simulink model "Model_pid_ff"  (R2024b)
settings: Solver=VariableStepAuto  StartTime=0.0  StopTime=25  RelTol=1e-3
PostLoadFcn:
  | addpath(fileparts(fileparts(get_param(bdroot,'FileName'))));
StartFcn:
  |    addpath(fullfile(fileparts(get_param(bdroot,'FileName')),'..','scripts'));
  |    run_and_save_deferred(bdroot, 'start');
StopFcn:
  |    addpath(fullfile(fileparts(get_param(bdroot,'FileName')),'..','scripts'));
  |    run_and_save_deferred(bdroot, 'stop');
undefined symbols (not defined in the file): k_3165_load, k_3166_load, kd_3165, kd_3166, ki_3165, ki_3166, kp_3165, kp_3166, tau_3165_load, tau_3166_load, Td_3165, Td_3166, Vc_3165, Vc_3166, w_eps, X, Y, Z
libraries: sm_lib x13, nesl_utility x5, slpidlib x2
settings Model: Creator=Student  LastModifiedBy=ricca

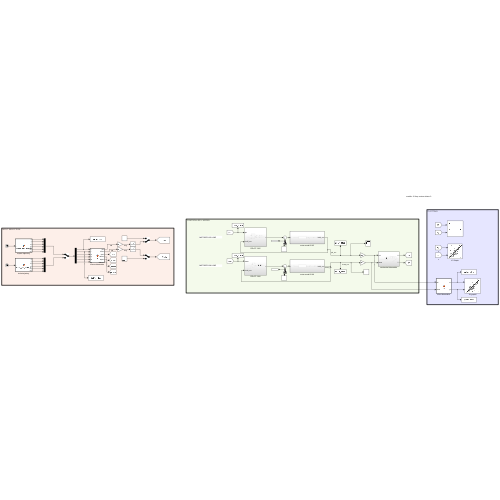
[thumbnail: Simulink's stored preview of the top-level diagram]
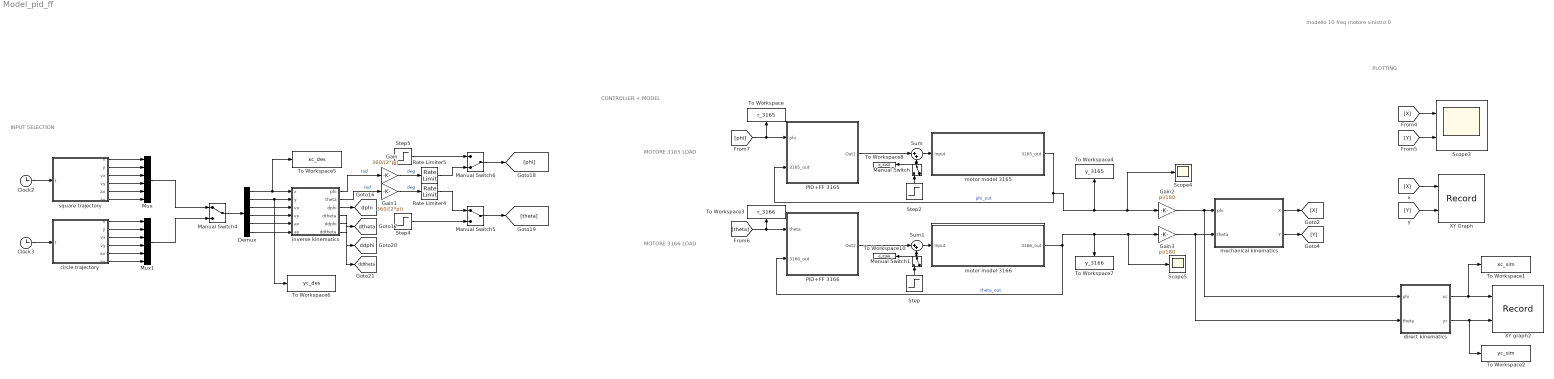
== system Model_pid_ff ==
  note: modello 10 freq motore sinistro 0
  note: PLOTTING
  note: INPUT SELECTION
  note: MOTORE 3166 LOAD
  note: CONTROLLER + MODEL
  note: MOTORE 3165 LOAD
  Clock2 : Clock
  Clock3 : Clock
  Demux : Demux  Outputs=6
  Gain : Gain  Gain=360/(2*pi)
  Gain1 : Gain  Gain=360/(2*pi)
  Gain2 : Gain  Gain=pi/180
  Gain3 : Gain  Gain=pi/180
  Manual Switch : ManualSwitch  CurrentSetting=0
  Manual Switch1 : ManualSwitch  CurrentSetting=0
  Manual Switch4 : ManualSwitch
  Manual Switch5 : ManualSwitch
  Manual Switch6 : ManualSwitch  CurrentSetting=0
  Mux : Mux  Inputs=6
  Mux1 : Mux  Inputs=6
  PID+FF 3165 : Subsystem
  PID+FF 3166 : Subsystem
  Rate Limiter4 : RateLimiter  RisingSlewLimit=100  FallingSlewLimit=-100  SampleTimeMode=inherited
  Rate Limiter5 : RateLimiter  RisingSlewLimit=100  FallingSlewLimit=-100  SampleTimeMode=inherited
  Scope3 : Scope  NumInputPorts=2
  Scope4 : Scope
  Scope5 : Scope
  Step : Step  Time=5  After=0.5  SampleTime=0
  Step2 : Step  Time=5  After=0.5  SampleTime=0
  Step4 : Step  After=10  SampleTime=0
  Step5 : Step  After=10  SampleTime=0
  Sum : Sum  Inputs=|++
  Sum1 : Sum  Inputs=|++
  To Workspace : ToWorkspace  VariableName=r_3165  SaveFormat=Timeseries  SampleTime=0.002
  To Workspace1 : ToWorkspace  VariableName=xc_sim  SaveFormat=Timeseries  SampleTime=0.002
  To Workspace10 : ToWorkspace  VariableName=d_3166  SaveFormat=Timeseries  SampleTime=-1
  To Workspace2 : ToWorkspace  VariableName=yc_sim  SaveFormat=Timeseries  SampleTime=0.002
  To Workspace3 : ToWorkspace  VariableName=r_3166  SaveFormat=Timeseries  SampleTime=0.002
  To Workspace4 : ToWorkspace  VariableName=y_3165  SaveFormat=Timeseries  SampleTime=0.002
  To Workspace5 : ToWorkspace  VariableName=xc_des  SaveFormat=Timeseries  SampleTime=0.002
  To Workspace6 : ToWorkspace  VariableName=yc_des  SaveFormat=Timeseries  SampleTime=0.002
  To Workspace7 : ToWorkspace  VariableName=y_3166  SaveFormat=Timeseries  SampleTime=0.002
  To Workspace8 : ToWorkspace  VariableName=d_3165  SaveFormat=Timeseries  SampleTime=-1
  XY Graph : Record  FileSettingsInternal="{\"entries\":[{\"content\":{\"excelSettings\":{\"content\":{},\"type\":\"Streamout.ExcelSettings\"}},\"type\":\"Streamout.FileSettingStorage\",\"uuid\":\"\"}],\"packageUris\":[\"http:\\/\\/schema.mathworks.com\\/mf0\\/streamout_blocks\\/R2020a\"],\"version\":\"1.0\"}"  Layout=[1 1]  SignalsInternal="{\"entries\":[{\"content\":{\"signals\":[{\"content\":{\"blockPath\":[],\"dimensions\":[1],\"domain\":\"\",\"lineColor\":\"#a2142f\",\"plots\":[ 1 ],\"port\":1,\"sid\":[\"\"],\"signalID\":1,\"signalName\":\"x\"},\"type\":\"RecordBlkView.Signal\",\"uuid\":\"\"},{\"content\":{\"blockPath\":[],\"dimensions\":[1],\"domain\":\"\",\"lineColor\":\"#139fff\",\"plots\":[ 1 ],\"port\":2,\"sid\":[\"\"],\"signalID\":2,\"signalName\":\"y\"},\"type\":\"RecordBlkView.Signal\",\"uuid\":\"\"}]},\"type\":\"RecordBlkView.InputSignals\",\"uuid\":\"\"}],\"packageUris\":[\"http:\\/\\/schema.mathworks.com\\/mf0\\/streamout_blocks\\/R2020a\"],\"version\":\"1.0\"}"  VisualizationBindings="{\"xyplotplugin\":{\"info\":[{\"series\":[{\"bindingParametersList\":[{\"parameter\":\"X-Axis\",\"signalID\":1,\"signalName\":\"x\"},{\"parameter\":\"Y-Axis\",\"signalID\":2,\"signalName\":\"y\"}],\"seriesID\":0}],\"subplotID\":1}]}}"  CompatibilityTag=XY
  XY graph2 : Record  FileSettingsInternal="{\"entries\":[{\"content\":{\"excelSettings\":{\"content\":{},\"type\":\"Streamout.ExcelSettings\"}},\"type\":\"Streamout.FileSettingStorage\",\"uuid\":\"\"}],\"packageUris\":[\"http:\\/\\/schema.mathworks.com\\/mf0\\/streamout_blocks\\/R2020a\"],\"version\":\"1.0\"}"  Layout=[1 1]  SignalsInternal="{\"entries\":[{\"content\":{\"signals\":[{\"content\":{\"blockPath\":[],\"dimensions\":[1],\"domain\":\"\",\"lineColor\":\"#64d413\",\"lineWidth\":2,\"port\":1,\"sid\":[\"\"],\"signalID\":1,\"signalName\":\"direct kinematics:1\"},\"type\":\"RecordBlkView.Signal\",\"uuid\":\"\"},{\"content\":{\"blockPath\":[],\"dimensions\":[1],\"domain\":\"\",\"lineColor\":\"#ff13a6\",\"lineWidth\":2,\"port\":2,\"sid\":[\"\"],\"signalID\":2,\"signalName\":\"direct kinematics:2\"},\"type\":\"RecordBlkView.Signal\",\"uuid\":\"\"}]},\"type\":\"RecordBlkView.InputSignals\",\"uuid\":\"\"}],\"packageUris\":[\"http:\\/\\/schema.mathworks.com\\/mf0\\/streamout_blocks\\/R2020a\"],\"version\":\"1.0\"}"  VisualizationBindings="{\"xyplotplugin\":{\"info\":[{\"series\":[],\"subplotID\":1}]}}"  CompatibilityTag=XY
  circle trajectory : MATLAB Function  TreatAsAtomicUnit=on
  direct kinematics : MATLAB Function  TreatAsAtomicUnit=on
  inverse kinematics : MATLAB Function  TreatAsAtomicUnit=on  SystemSampleTime=0.002
  mechanical kinematics : Subsystem
  motor model 3165 : Subsystem
  motor model 3166 : Subsystem
  square trajectory : MATLAB Function  TreatAsAtomicUnit=on
  tag scope: ddphi=global, ddtheta=global, dphi=global, dtheta=global
  wires:
  Sum/1 -> motor model 3165/1(Input)
  Sum1/1 -> motor model 3166/1(Input)
  Gain3/1 -> mechanical kinematics/2(theta), direct kinematics/2(theta)
  Rate Limiter5/1 -> Manual Switch6/2
  Demux/1 -> inverse kinematics/1(x), To Workspace5/1
  [Y] -> Scope3/2
  Manual Switch5/1 -> [theta]
  circle trajectory/6(ay) -> Mux1/6
  [Y] -> XY Graph/2
  PID+FF 3166/1(Out2) -> Sum1/1
  Clock3/1 -> circle trajectory/1(t)
  Manual Switch6/1 -> [phi]
  direct kinematics/1(xc) -> To Workspace1/1, XY graph2/1
  Mux1/1 -> Manual Switch4/2
  square trajectory/2(y) -> Mux/2
  inverse kinematics/3(dphi) -> [dphi]
  square trajectory/1(x) -> Mux/1
  Clock2/1 -> square trajectory/1(t)
  [X] -> XY Graph/1
  circle trajectory/2(y) -> Mux1/2
  inverse kinematics/4(dtheta) -> [dtheta]
  [theta] -> To Workspace3/1, PID+FF 3166/1(theta)
  square trajectory/6(ay) -> Mux/6
  Step4/1 -> Manual Switch5/2
  circle trajectory/3(vx) -> Mux1/3
  Mux/1 -> Manual Switch4/1
  inverse kinematics/1(phi) -> Gain/1  "rad"
  [phi] -> To Workspace/1, PID+FF 3165/1(phi)
  motor model 3165/1(3165_out) -> PID+FF 3165/2(3165_out), Gain2/1, Scope4/1, To Workspace4/1  "phi_out"
  circle trajectory/4(vy) -> Mux1/4
  Demux/2 -> To Workspace6/1, inverse kinematics/2(y)
  circle trajectory/5(ax) -> Mux1/5
  inverse kinematics/6(ddtheta) -> [ddtheta]
  Gain1/1 -> Rate Limiter4/1  "deg"
  motor model 3166/1(3166_out) -> PID+FF 3166/2(3166_out), To Workspace7/1, Gain3/1, Scope5/1  "theta_out"
  Gain2/1 -> direct kinematics/1(phi), mechanical kinematics/1(phi)
  inverse kinematics/2(theta) -> Gain1/1  "rad"
  inverse kinematics/5(ddphi) -> [ddphi]
  mechanical kinematics/2(Y) -> [Y]
  Step5/1 -> Manual Switch6/1
  Demux/6 -> inverse kinematics/6(ay)
  Demux/4 -> inverse kinematics/4(vy)
  Gain/1 -> Rate Limiter5/1  "deg"
  direct kinematics/2(yc) -> To Workspace2/1, XY graph2/2
  Demux/3 -> inverse kinematics/3(vx)
  square trajectory/3(vx) -> Mux/3
  circle trajectory/1(x) -> Mux1/1
  [X] -> Scope3/1
  PID+FF 3165/1(Out1) -> Sum/1
  Demux/5 -> inverse kinematics/5(ax)
  square trajectory/5(ax) -> Mux/5
  mechanical kinematics/1(X) -> [X]
  Rate Limiter4/1 -> Manual Switch5/1
  Manual Switch4/1 -> Demux/1
  square trajectory/4(vy) -> Mux/4
  Step2/1 -> Manual Switch/1
  Manual Switch/1 -> Sum/2, To Workspace8/1
  Step/1 -> Manual Switch1/1
  Manual Switch1/1 -> Sum1/2, To Workspace10/1

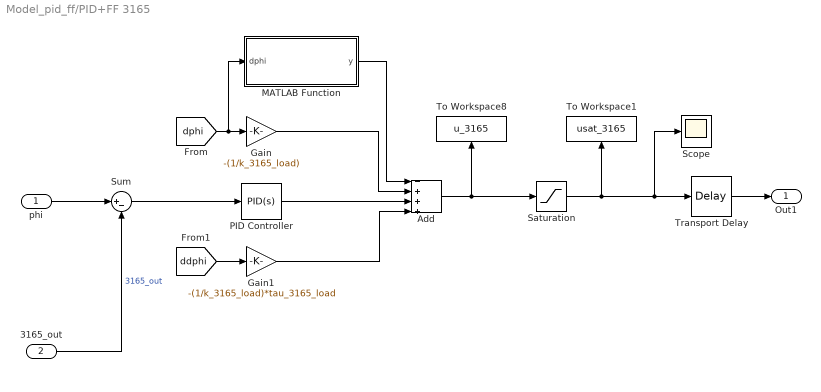
== system Model_pid_ff/PID+FF 3165 ==
  phi : Inport
  3165_out : Inport  Port=2
  Add : Sum  Inputs=-+++
  Gain : Gain  Gain=-(1/k_3165_load)
  Gain1 : Gain  Gain=-(1/k_3165_load)*tau_3165_load
  MATLAB Function : MATLAB Function  TreatAsAtomicUnit=on
  PID Controller : slpidlib/PID Controller  Controller=PID  Form=Parallel  TimeDomain=Continuous-time  UseExternalTs=off  SampleTime=-1  IntegratorMethod=Forward Euler  FilterMethod=Forward Euler  ControllerParametersSource=internal  P=kp_3165  I=ki_3165  UseKiTs=off  D=kd_3165  UseExternalDerivativeSource=off  N=100  UseFilter=on  TunerSelectOption=Transfer Function Based (PID Tuner App)  InitialConditionSource=internal  InitialConditionForIntegrator=0  InitialConditionForFilter=0  DifferentiatorICPrevScaledInput=0  ExternalReset=none  TrackingMode=off  Kt=1  LimitOutput=off  SatLimitsSource=internal  UpperSaturationLimit=inf  LowerSaturationLimit=-inf  LinearizeAsGain=on  AntiWindupMode=none  Kb=1  LimitIntegrator=off  UpperIntegratorSaturationLimit=inf  LowerIntegratorSaturationLimit=-inf  POutMin=[]  POutMax=[]  IOutMin=[]  IOutMax=[]  DOutMin=[]  DOutMax=[]  NOutMin=[]  NOutMax=[]  SumOutMin=[]  SumOutMax=[]  SaturationOutMin=[]  SaturationOutMax=[]  PParamMin=[]  PParamMax=[]  IParamMin=[]  IParamMax=[]  DParamMin=[]  DParamMax=[]  NParamMin=[]  NParamMax=[]  KbParamMin=[]  KbParamMax=[]  KtParamMin=[]  KtParamMax=[]  KbOutMin=[]  KbOutMax=[]  KtOutMin=[]  KtOutMax=[]  IntegratorOutMin=[]  IntegratorOutMax=[]  FilterOutMin=[]  FilterOutMax=[]  SumI1OutMin=[]  SumI1OutMax=[]  SumI2OutMin=[]  SumI2OutMax=[]  SumI3OutMin=[]  SumI3OutMax=[]  SumI4OutMin=[]  SumI4OutMax=[]  SumDOutMin=[]  SumDOutMax=[]  DifferentiatorOutMin=[]  DifferentiatorOutMax=[]  FilterDiffOutCoefMin=[]  FilterDiffOutCoefMax=[]  ReciprocalOutMin=[]  ReciprocalOutMax=[]  SumDenOutMin=[]  SumDenOutMax=[]  SumNumOutMin=[]  SumNumOutMax=[]  DivideOutMin=[]  DivideOutMax=[]  UdiffTsProdOutMin=[]  UdiffTsProdOutMax=[]  NTsProdOutMin=[]  NTsProdOutMax=[]  UintegralTsProdOutMin=[]  UintegralTsProdOutMax=[]  UngainTsProdOutMin=[]  UngainTsProdOutMax=[]  ClampingZeroOutDataTypeStr=Inherit: Inherit via back propagation  ClampingZeroOutMin=[]  ClampingZeroOutMax=[]  FilterDenConstantOutDataTypeStr=Inherit: Inherit via back propagation  FilterDenConstantOutMin=[]  FilterDenConstantOutMax=[]  PCopyOutDataTypeStr=Inherit: Inherit via back propagation  PCopyOutMin=[]  PCopyOutMax=[]  NCopyOutDataTypeStr=Inherit: Inherit via back propagation  NCopyOutMin=[]  NCopyOutMax=[]  IntegratorContinuousStateAttributes=''  IntegratorStateMustResolveToSignalObject=off  IntegratorRTWStateStorageClass=Auto  FilterContinuousStateAttributes=''  FilterStateMustResolveToSignalObject=off  FilterRTWStateStorageClass=Auto  ParallelPVariant=InternalParameters  IdealPVariant=Disabled  IVariant=InternalParameters  DVariant=InternalParameters  IntegratorVariant=Continuous  SatVariant=Disabled  AWVariant=Passthrough  PCopyVariant=Disabled  TRVariant=Disabled  FdbkBlocksVariant=Forward  IdealPFdbkVariant=Disabled  SatFdbkVariant=Disabled  DerivativeFilterVariant=ContFilter  NVariant=InternalParameters  NCopyVariant=Disabled  FilterICVariant=InternalICsFilter  IntegratorICVariant=InternalICs  ExternalResetVariant=Disabled  TRSumVariant=Passthrough  SumFdbkVariant=Disabled  SumVariant=Sum_PID  TsampFilterVariant=InternalTs  TsampNgainVariant=Passthrough  TsampIntegralVariant=Disabled_SignalSpec  ExternalSaturationOutDataTypeStr=Inherit: Same as second input  DerivativeSourceVariant=ErrorSignal  PreIntVariant=InternalPreInt
  Saturation : Saturate  UpperLimit=6  LowerLimit=-6
  Scope : Scope
  Sum : Sum  Inputs=|+-
  To Workspace1 : ToWorkspace  VariableName=usat_3165  SaveFormat=Timeseries  SampleTime=0.002
  To Workspace8 : ToWorkspace  VariableName=u_3165  SaveFormat=Timeseries  SampleTime=0.002
  Transport Delay : TransportDelay  DelayTime=Td_3165  PadeOrder=2
  Out1 : Outport
  wires:
  3165_out/1 -> Sum/2  "3165_out"
  [ddphi] -> Gain1/1
  phi/1 -> Sum/1
  Sum/1 -> PID Controller/1
  Add/1 -> Saturation/1, To Workspace8/1
  Saturation/1 -> Scope/1, Transport Delay/1, To Workspace1/1
  [dphi] -> MATLAB Function/1(dphi), Gain/1
  MATLAB Function/1(y) -> Add/1
  Gain/1 -> Add/2
  PID Controller/1 -> Add/3
  Gain1/1 -> Add/4
  Transport Delay/1 -> Out1/1

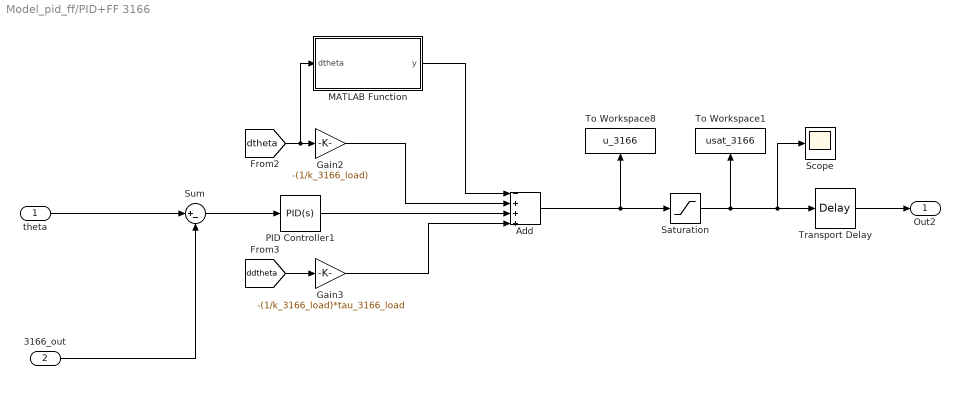
== system Model_pid_ff/PID+FF 3166 ==
  theta : Inport
  3166_out : Inport  Port=2
  Add : Sum  Inputs=-+++
  Gain2 : Gain  Gain=-(1/k_3166_load)
  Gain3 : Gain  Gain=-(1/k_3166_load)*tau_3166_load
  MATLAB Function : MATLAB Function  TreatAsAtomicUnit=on
  PID Controller1 : slpidlib/PID Controller  Controller=PID  Form=Parallel  TimeDomain=Continuous-time  UseExternalTs=off  SampleTime=-1  IntegratorMethod=Forward Euler  FilterMethod=Forward Euler  ControllerParametersSource=internal  P=kp_3166  I=ki_3166  UseKiTs=off  D=kd_3166  UseExternalDerivativeSource=off  N=100  UseFilter=on  TunerSelectOption=Transfer Function Based (PID Tuner App)  InitialConditionSource=internal  InitialConditionForIntegrator=0  InitialConditionForFilter=0  DifferentiatorICPrevScaledInput=0  ExternalReset=none  TrackingMode=off  Kt=1  LimitOutput=off  SatLimitsSource=internal  UpperSaturationLimit=inf  LowerSaturationLimit=-inf  LinearizeAsGain=on  AntiWindupMode=none  Kb=1  LimitIntegrator=off  UpperIntegratorSaturationLimit=inf  LowerIntegratorSaturationLimit=-inf  POutMin=[]  POutMax=[]  IOutMin=[]  IOutMax=[]  DOutMin=[]  DOutMax=[]  NOutMin=[]  NOutMax=[]  SumOutMin=[]  SumOutMax=[]  SaturationOutMin=[]  SaturationOutMax=[]  PParamMin=[]  PParamMax=[]  IParamMin=[]  IParamMax=[]  DParamMin=[]  DParamMax=[]  NParamMin=[]  NParamMax=[]  KbParamMin=[]  KbParamMax=[]  KtParamMin=[]  KtParamMax=[]  KbOutMin=[]  KbOutMax=[]  KtOutMin=[]  KtOutMax=[]  IntegratorOutMin=[]  IntegratorOutMax=[]  FilterOutMin=[]  FilterOutMax=[]  SumI1OutMin=[]  SumI1OutMax=[]  SumI2OutMin=[]  SumI2OutMax=[]  SumI3OutMin=[]  SumI3OutMax=[]  SumI4OutMin=[]  SumI4OutMax=[]  SumDOutMin=[]  SumDOutMax=[]  DifferentiatorOutMin=[]  DifferentiatorOutMax=[]  FilterDiffOutCoefMin=[]  FilterDiffOutCoefMax=[]  ReciprocalOutMin=[]  ReciprocalOutMax=[]  SumDenOutMin=[]  SumDenOutMax=[]  SumNumOutMin=[]  SumNumOutMax=[]  DivideOutMin=[]  DivideOutMax=[]  UdiffTsProdOutMin=[]  UdiffTsProdOutMax=[]  NTsProdOutMin=[]  NTsProdOutMax=[]  UintegralTsProdOutMin=[]  UintegralTsProdOutMax=[]  UngainTsProdOutMin=[]  UngainTsProdOutMax=[]  ClampingZeroOutDataTypeStr=Inherit: Inherit via back propagation  ClampingZeroOutMin=[]  ClampingZeroOutMax=[]  FilterDenConstantOutDataTypeStr=Inherit: Inherit via back propagation  FilterDenConstantOutMin=[]  FilterDenConstantOutMax=[]  PCopyOutDataTypeStr=Inherit: Inherit via back propagation  PCopyOutMin=[]  PCopyOutMax=[]  NCopyOutDataTypeStr=Inherit: Inherit via back propagation  NCopyOutMin=[]  NCopyOutMax=[]  IntegratorContinuousStateAttributes=''  IntegratorStateMustResolveToSignalObject=off  IntegratorRTWStateStorageClass=Auto  FilterContinuousStateAttributes=''  FilterStateMustResolveToSignalObject=off  FilterRTWStateStorageClass=Auto  ParallelPVariant=InternalParameters  IdealPVariant=Disabled  IVariant=InternalParameters  DVariant=InternalParameters  IntegratorVariant=Continuous  SatVariant=Disabled  AWVariant=Passthrough  PCopyVariant=Disabled  TRVariant=Disabled  FdbkBlocksVariant=Forward  IdealPFdbkVariant=Disabled  SatFdbkVariant=Disabled  DerivativeFilterVariant=ContFilter  NVariant=InternalParameters  NCopyVariant=Disabled  FilterICVariant=InternalICsFilter  IntegratorICVariant=InternalICs  ExternalResetVariant=Disabled  TRSumVariant=Passthrough  SumFdbkVariant=Disabled  SumVariant=Sum_PID  TsampFilterVariant=InternalTs  TsampNgainVariant=Passthrough  TsampIntegralVariant=Disabled_SignalSpec  ExternalSaturationOutDataTypeStr=Inherit: Same as second input  DerivativeSourceVariant=ErrorSignal  PreIntVariant=InternalPreInt
  Saturation : Saturate  UpperLimit=6  LowerLimit=-6
  Scope : Scope
  Sum : Sum  Inputs=|+-
  To Workspace1 : ToWorkspace  VariableName=usat_3166  SaveFormat=Timeseries  SampleTime=0.002
  To Workspace8 : ToWorkspace  VariableName=u_3166  SaveFormat=Timeseries  SampleTime=0.002
  Transport Delay : TransportDelay  DelayTime=Td_3166  PadeOrder=2
  Out2 : Outport
  wires:
  3166_out/1 -> Sum/2
  [ddtheta] -> Gain3/1
  Sum/1 -> PID Controller1/1
  [dtheta] -> MATLAB Function/1(dtheta), Gain2/1
  Add/1 -> Saturation/1, To Workspace8/1
  theta/1 -> Sum/1
  Saturation/1 -> Scope/1, Transport Delay/1, To Workspace1/1
  MATLAB Function/1(y) -> Add/1
  Gain2/1 -> Add/2
  PID Controller1/1 -> Add/3
  Gain3/1 -> Add/4
  Transport Delay/1 -> Out2/1

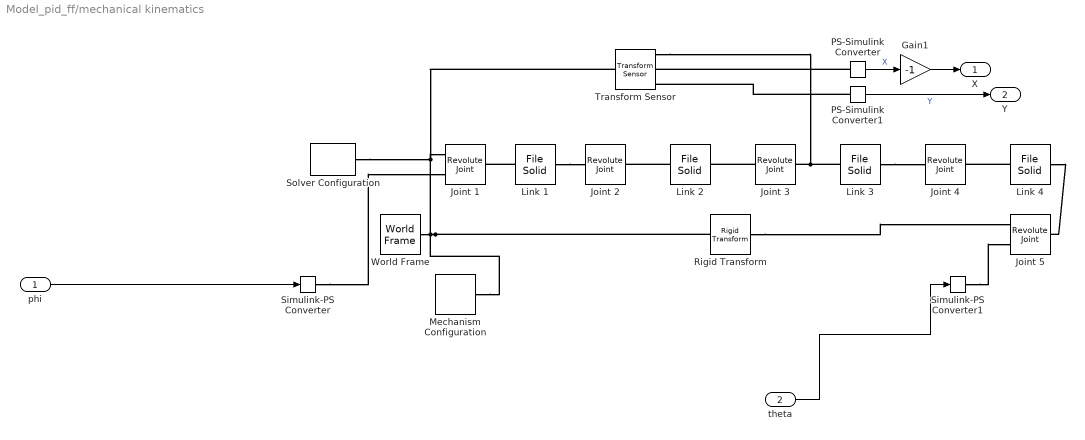
== system Model_pid_ff/mechanical kinematics ==
  phi : Inport
  theta : Inport  Port=2
  Gain1 : Gain  Gain=-1
  Joint 1 : sm_lib/Joints/Revolute Joint  JointMode=Normal  CompositeWrenchDir=FollowerOnBase  CompositeWrenchFrame=BaseFrame  SenseConstraintForce=off  SenseConstraintTorque=off  SenseTotalForce=off  SenseTotalTorque=off  PositionTargetSpecify=off  PositionTargetPriority=High  PositionTargetValue=0  PositionTargetValueUnits=deg  VelocityTargetSpecify=off  VelocityTargetPriority=High  VelocityTargetValue=0  VelocityTargetValueUnits=deg/s  EquilibriumPosition=0  EquilibriumPositionUnits=deg  SpringStiffness=0  SpringStiffnessUnits=N*m/deg  DampingCoefficient=0  DampingCoefficientUnits=N*m/(deg/s)  LowerLimitSpecify=off  LowerLimitBound=-90  LowerLimitBoundUnits=deg  LowerLimitStiffness=1e4  LowerLimitStiffnessUnits=N*m/deg  LowerLimitDamping=10  LowerLimitDampingUnits=N*m/(deg/s)  LowerLimitTransitionRegionWidth=0.1  LowerLimitTransitionRegionWidthUnits=deg  UpperLimitSpecify=off  UpperLimitBound=90  UpperLimitBoundUnits=deg  UpperLimitStiffness=1e4  UpperLimitStiffnessUnits=N*m/deg  UpperLimitDamping=10  UpperLimitDampingUnits=N*m/(deg/s)  UpperLimitTransitionRegionWidth=0.1  UpperLimitTransitionRegionWidthUnits=deg  TorqueActuationMode=ComputedTorque  MotionActuationMode=InputMotion  SensePosition=off  SenseVelocity=off  SenseAcceleration=off  SenseTorqueForce=off  SenseLowerLimitTorqueForce=off  SenseUpperLimitTorqueForce=off
  Joint 2 : sm_lib/Joints/Revolute Joint  JointMode=Normal  CompositeWrenchDir=FollowerOnBase  CompositeWrenchFrame=BaseFrame  SenseConstraintForce=off  SenseConstraintTorque=off  SenseTotalForce=off  SenseTotalTorque=off  PositionTargetSpecify=off  PositionTargetPriority=High  PositionTargetValue=90  PositionTargetValueUnits=deg  VelocityTargetSpecify=off  VelocityTargetPriority=High  VelocityTargetValue=0  VelocityTargetValueUnits=deg/s  EquilibriumPosition=0  EquilibriumPositionUnits=deg  SpringStiffness=0  SpringStiffnessUnits=N*m/deg  DampingCoefficient=0  DampingCoefficientUnits=N*m/(deg/s)  LowerLimitSpecify=off  LowerLimitBound=-90  LowerLimitBoundUnits=deg  LowerLimitStiffness=1e4  LowerLimitStiffnessUnits=N*m/deg  LowerLimitDamping=10  LowerLimitDampingUnits=N*m/(deg/s)  LowerLimitTransitionRegionWidth=0.1  LowerLimitTransitionRegionWidthUnits=deg  UpperLimitSpecify=off  UpperLimitBound=90  UpperLimitBoundUnits=deg  UpperLimitStiffness=1e4  UpperLimitStiffnessUnits=N*m/deg  UpperLimitDamping=10  UpperLimitDampingUnits=N*m/(deg/s)  UpperLimitTransitionRegionWidth=0.1  UpperLimitTransitionRegionWidthUnits=deg  TorqueActuationMode=NoTorque  MotionActuationMode=ComputedMotion  SensePosition=off  SenseVelocity=off  SenseAcceleration=off  SenseTorqueForce=off  SenseLowerLimitTorqueForce=off  SenseUpperLimitTorqueForce=off
  Joint 3 : sm_lib/Joints/Revolute Joint  JointMode=Normal  CompositeWrenchDir=FollowerOnBase  CompositeWrenchFrame=BaseFrame  SenseConstraintForce=off  SenseConstraintTorque=off  SenseTotalForce=off  SenseTotalTorque=off  PositionTargetSpecify=off  PositionTargetPriority=High  PositionTargetValue=0  PositionTargetValueUnits=deg  VelocityTargetSpecify=off  VelocityTargetPriority=High  VelocityTargetValue=0  VelocityTargetValueUnits=deg/s  EquilibriumPosition=0  EquilibriumPositionUnits=deg  SpringStiffness=0  SpringStiffnessUnits=N*m/deg  DampingCoefficient=0  DampingCoefficientUnits=N*m/(deg/s)  LowerLimitSpecify=off  LowerLimitBound=-90  LowerLimitBoundUnits=deg  LowerLimitStiffness=1e4  LowerLimitStiffnessUnits=N*m/deg  LowerLimitDamping=10  LowerLimitDampingUnits=N*m/(deg/s)  LowerLimitTransitionRegionWidth=0.1  LowerLimitTransitionRegionWidthUnits=deg  UpperLimitSpecify=off  UpperLimitBound=90  UpperLimitBoundUnits=deg  UpperLimitStiffness=1e4  UpperLimitStiffnessUnits=N*m/deg  UpperLimitDamping=10  UpperLimitDampingUnits=N*m/(deg/s)  UpperLimitTransitionRegionWidth=0.1  UpperLimitTransitionRegionWidthUnits=deg  TorqueActuationMode=NoTorque  MotionActuationMode=ComputedMotion  SensePosition=off  SenseVelocity=off  SenseAcceleration=off  SenseTorqueForce=off  SenseLowerLimitTorqueForce=off  SenseUpperLimitTorqueForce=off
  Joint 4 : sm_lib/Joints/Revolute Joint  JointMode=Normal  CompositeWrenchDir=FollowerOnBase  CompositeWrenchFrame=BaseFrame  SenseConstraintForce=off  SenseConstraintTorque=off  SenseTotalForce=off  SenseTotalTorque=off  PositionTargetSpecify=off  PositionTargetPriority=High  PositionTargetValue=0  PositionTargetValueUnits=deg  VelocityTargetSpecify=off  VelocityTargetPriority=High  VelocityTargetValue=0  VelocityTargetValueUnits=deg/s  EquilibriumPosition=0  EquilibriumPositionUnits=deg  SpringStiffness=0  SpringStiffnessUnits=N*m/deg  DampingCoefficient=0  DampingCoefficientUnits=N*m/(deg/s)  LowerLimitSpecify=off  LowerLimitBound=-90  LowerLimitBoundUnits=deg  LowerLimitStiffness=1e4  LowerLimitStiffnessUnits=N*m/deg  LowerLimitDamping=10  LowerLimitDampingUnits=N*m/(deg/s)  LowerLimitTransitionRegionWidth=0.1  LowerLimitTransitionRegionWidthUnits=deg  UpperLimitSpecify=off  UpperLimitBound=90  UpperLimitBoundUnits=deg  UpperLimitStiffness=1e4  UpperLimitStiffnessUnits=N*m/deg  UpperLimitDamping=10  UpperLimitDampingUnits=N*m/(deg/s)  UpperLimitTransitionRegionWidth=0.1  UpperLimitTransitionRegionWidthUnits=deg  TorqueActuationMode=NoTorque  MotionActuationMode=ComputedMotion  SensePosition=off  SenseVelocity=off  SenseAcceleration=off  SenseTorqueForce=off  SenseLowerLimitTorqueForce=off  SenseUpperLimitTorqueForce=off
  Joint 5 : sm_lib/Joints/Revolute Joint  JointMode=Normal  CompositeWrenchDir=FollowerOnBase  CompositeWrenchFrame=BaseFrame  SenseConstraintForce=off  SenseConstraintTorque=off  SenseTotalForce=off  SenseTotalTorque=off  PositionTargetSpecify=off  PositionTargetPriority=High  PositionTargetValue=0  PositionTargetValueUnits=deg  VelocityTargetSpecify=off  VelocityTargetPriority=High  VelocityTargetValue=0  VelocityTargetValueUnits=deg/s  EquilibriumPosition=0  EquilibriumPositionUnits=deg  SpringStiffness=0  SpringStiffnessUnits=N*m/deg  DampingCoefficient=0  DampingCoefficientUnits=N*m/(deg/s)  LowerLimitSpecify=off  LowerLimitBound=-90  LowerLimitBoundUnits=deg  LowerLimitStiffness=1e4  LowerLimitStiffnessUnits=N*m/deg  LowerLimitDamping=10  LowerLimitDampingUnits=N*m/(deg/s)  LowerLimitTransitionRegionWidth=0.1  LowerLimitTransitionRegionWidthUnits=deg  UpperLimitSpecify=off  UpperLimitBound=90  UpperLimitBoundUnits=deg  UpperLimitStiffness=1e4  UpperLimitStiffnessUnits=N*m/deg  UpperLimitDamping=10  UpperLimitDampingUnits=N*m/(deg/s)  UpperLimitTransitionRegionWidth=0.1  UpperLimitTransitionRegionWidthUnits=deg  TorqueActuationMode=ComputedTorque  MotionActuationMode=InputMotion  SensePosition=off  SenseVelocity=off  SenseAcceleration=off  SenseTorqueForce=off  SenseLowerLimitTorqueForce=off  SenseUpperLimitTorqueForce=off
  Link 1 : sm_lib/Body Elements/File Solid  ExtGeomFileName=link.step  UnitType=FromFile  ExtGeomFileUnits=m  StepReaderType=HEX  ExportConvexHullGeometry=off  InertiaType=CalculateFromGeometry  BasedOnType=Mass  Density=1000  DensityUnits=kg/m^3  Mass=0.065  MassUnits=kg  CenterOfMass=[0 0 0]  CenterOfMassUnits=m  MomentsOfInertia=[1 1 1]  MomentsOfInertiaUnits=kg*m^2  ProductsOfInertia=[0 0 0]  ProductsOfInertiaUnits=kg*m^2  GraphicType=FromGeometry  MarkerShape=Sphere  MarkerSize=10  GraphicVisPropType=SimpleVisualProperties  GraphicDiffuseColor=[0.5 0.5 0.5]  GraphicOpacity=1  GraphicSpecularColor=[0.5 0.5 0.5 1.0]  GraphicAmbientColor=[0.15 0.15 0.15 1.0]  GraphicEmissiveColor=[0.0 0.0 0.0 1.0]  GraphicShininess=75  DoExposeReferenceFrame=off  SerializedFrames=<Frames><Frame><Id>Frame1</Id><Value><Name>F1</Name><Origin><Source>GeometricFeature</Source><FeatureName>cylindrical surface 1</FeatureName></Origin><PrimaryAxis><DefinedDirection>+Z</DefinedDirection><Source>ReferenceFrame</Source><SourceDirection>+Z</SourceDirection><FeatureName></FeatureName></PrimaryAxis><SecondaryAxis><DefinedDirection>+Y</DefinedDirection><Source>ReferenceFrame</Source><SourceDirection>+X</SourceDirection><FeatureName></FeatureName></SecondaryAxis></Value></Frame><Frame><Id>Frame2</Id><Value><Name>F2</Name><Origin><Source>GeometricFeature</Source><FeatureName>cylindrical surface 2</FeatureName></Origin><PrimaryAxis><DefinedDirection>+Z</DefinedDirection><Source>ReferenceFrame</Source><SourceDirection>+Z</SourceDirection><FeatureName></FeatureName></PrimaryAxis><SecondaryAxis><DefinedDirection>+X</DefinedDirection><Source>ReferenceFrame</Source><SourceDirection>+X</SourceDirection><FeatureName></FeatureName></SecondaryAxis></Value></Frame></Frames>
  Link 2 : sm_lib/Body Elements/File Solid  ExtGeomFileName=link.step  UnitType=FromFile  ExtGeomFileUnits=m  StepReaderType=HEX  ExportConvexHullGeometry=off  InertiaType=CalculateFromGeometry  BasedOnType=Mass  Density=1000  DensityUnits=kg/m^3  Mass=0.065  MassUnits=kg  CenterOfMass=[0 0 0]  CenterOfMassUnits=m  MomentsOfInertia=[1 1 1]  MomentsOfInertiaUnits=kg*m^2  ProductsOfInertia=[0 0 0]  ProductsOfInertiaUnits=kg*m^2  GraphicType=FromGeometry  MarkerShape=Sphere  MarkerSize=10  GraphicVisPropType=SimpleVisualProperties  GraphicDiffuseColor=[0.5 0.5 0.5]  GraphicOpacity=1  GraphicSpecularColor=[0.5 0.5 0.5 1.0]  GraphicAmbientColor=[0.15 0.15 0.15 1.0]  GraphicEmissiveColor=[0.0 0.0 0.0 1.0]  GraphicShininess=75  DoExposeReferenceFrame=off  SerializedFrames=<Frames><Frame><Id>Frame1</Id><Value><Name>F1</Name><Origin><Source>GeometricFeature</Source><FeatureName>cylindrical surface 1</FeatureName></Origin><PrimaryAxis><DefinedDirection>+Z</DefinedDirection><Source>ReferenceFrame</Source><SourceDirection>+Z</SourceDirection><FeatureName></FeatureName></PrimaryAxis><SecondaryAxis><DefinedDirection>+X</DefinedDirection><Source>ReferenceFrame</Source><SourceDirection>+X</SourceDirection><FeatureName></FeatureName></SecondaryAxis></Value></Frame><Frame><Id>Frame2</Id><Value><Name>F2</Name><Origin><Source>GeometricFeature</Source><FeatureName>cylindrical surface 2</FeatureName></Origin><PrimaryAxis><DefinedDirection>+Z</DefinedDirection><Source>ReferenceFrame</Source><SourceDirection>+Z</SourceDirection><FeatureName></FeatureName></PrimaryAxis><SecondaryAxis><DefinedDirection>+X</DefinedDirection><Source>ReferenceFrame</Source><SourceDirection>+X</SourceDirection><FeatureName></FeatureName></SecondaryAxis></Value></Frame></Frames>
  Link 3 : sm_lib/Body Elements/File Solid  ExtGeomFileName=link.step  UnitType=FromFile  ExtGeomFileUnits=m  StepReaderType=HEX  ExportConvexHullGeometry=off  InertiaType=CalculateFromGeometry  BasedOnType=Mass  Density=1000  DensityUnits=kg/m^3  Mass=0.065  MassUnits=kg  CenterOfMass=[0 0 0]  CenterOfMassUnits=m  MomentsOfInertia=[1 1 1]  MomentsOfInertiaUnits=kg*m^2  ProductsOfInertia=[0 0 0]  ProductsOfInertiaUnits=kg*m^2  GraphicType=FromGeometry  MarkerShape=Sphere  MarkerSize=10  GraphicVisPropType=SimpleVisualProperties  GraphicDiffuseColor=[0.5 0.5 0.5]  GraphicOpacity=1  GraphicSpecularColor=[0.5 0.5 0.5 1.0]  GraphicAmbientColor=[0.15 0.15 0.15 1.0]  GraphicEmissiveColor=[0.0 0.0 0.0 1.0]  GraphicShininess=75  DoExposeReferenceFrame=off  SerializedFrames=<Frames><Frame><Id>Frame1</Id><Value><Name>F1</Name><Origin><Source>GeometricFeature</Source><FeatureName>cylindrical surface 1</FeatureName></Origin><PrimaryAxis><DefinedDirection>+Z</DefinedDirection><Source>ReferenceFrame</Source><SourceDirection>+Z</SourceDirection><FeatureName></FeatureName></PrimaryAxis><SecondaryAxis><DefinedDirection>+X</DefinedDirection><Source>ReferenceFrame</Source><SourceDirection>+X</SourceDirection><FeatureName></FeatureName></SecondaryAxis></Value></Frame><Frame><Id>Frame2</Id><Value><Name>F2</Name><Origin><Source>GeometricFeature</Source><FeatureName>cylindrical surface 2</FeatureName></Origin><PrimaryAxis><DefinedDirection>+Z</DefinedDirection><Source>ReferenceFrame</Source><SourceDirection>+Z</SourceDirection><FeatureName></FeatureName></PrimaryAxis><SecondaryAxis><DefinedDirection>+X</DefinedDirection><Source>ReferenceFrame</Source><SourceDirection>+X</SourceDirection><FeatureName></FeatureName></SecondaryAxis></Value></Frame></Frames>
  Link 4 : sm_lib/Body Elements/File Solid  ExtGeomFileName=link.step  UnitType=FromFile  ExtGeomFileUnits=m  StepReaderType=HEX  ExportConvexHullGeometry=off  InertiaType=CalculateFromGeometry  BasedOnType=Mass  Density=1000  DensityUnits=kg/m^3  Mass=0.065  MassUnits=kg  CenterOfMass=[0 0 0]  CenterOfMassUnits=m  MomentsOfInertia=[1 1 1]  MomentsOfInertiaUnits=kg*m^2  ProductsOfInertia=[0 0 0]  ProductsOfInertiaUnits=kg*m^2  GraphicType=FromGeometry  MarkerShape=Sphere  MarkerSize=10  GraphicVisPropType=SimpleVisualProperties  GraphicDiffuseColor=[0.5 0.5 0.5]  GraphicOpacity=1  GraphicSpecularColor=[0.5 0.5 0.5 1.0]  GraphicAmbientColor=[0.15 0.15 0.15 1.0]  GraphicEmissiveColor=[0.0 0.0 0.0 1.0]  GraphicShininess=75  DoExposeReferenceFrame=off  SerializedFrames=<Frames><Frame><Id>Frame1</Id><Value><Name>F1</Name><Origin><Source>GeometricFeature</Source><FeatureName>cylindrical surface 1</FeatureName></Origin><PrimaryAxis><DefinedDirection>+Z</DefinedDirection><Source>ReferenceFrame</Source><SourceDirection>+Z</SourceDirection><FeatureName></FeatureName></PrimaryAxis><SecondaryAxis><DefinedDirection>+X</DefinedDirection><Source>ReferenceFrame</Source><SourceDirection>+X</SourceDirection><FeatureName></FeatureName></SecondaryAxis></Value></Frame><Frame><Id>Frame2</Id><Value><Name>F2</Name><Origin><Source>GeometricFeature</Source><FeatureName>cylindrical surface 2</FeatureName></Origin><PrimaryAxis><DefinedDirection>+Z</DefinedDirection><Source>ReferenceFrame</Source><SourceDirection>+Z</SourceDirection><FeatureName></FeatureName></PrimaryAxis><SecondaryAxis><DefinedDirection>+X</DefinedDirection><Source>ReferenceFrame</Source><SourceDirection>+X</SourceDirection><FeatureName></FeatureName></SecondaryAxis></Value></Frame></Frames>
  Mechanism Configuration : sm_lib/Utilities/Mechanism Configuration  UniformGravity=Constant  GravityVector=[0 0 -9.80665]  GravityVectorUnits=m/s^2  LinearizationDelta=0.001  JointModeTransitionNonlinearIterations=2
  PS-Simulink Converter : nesl_utility/PS-Simulink Converter  PhysicalDomain=network_engine_domain  SubClassName=ps_output  LeftPortType=input  RightPortType=output  PseudoPeriodic=off  Frequencies=[]  VectorFormat=inherit  Unit=inherit  AffineConversion=off
  PS-Simulink Converter1 : nesl_utility/PS-Simulink Converter  PhysicalDomain=network_engine_domain  SubClassName=ps_output  LeftPortType=input  RightPortType=output  PseudoPeriodic=off  Frequencies=[]  VectorFormat=inherit  Unit=inherit  AffineConversion=off
  Rigid Transform : sm_lib/Frames and Transforms/Rigid Transform  RotationMethod=None  FollAlignAxisA=+X  BaseAlignAxisA=+Y  FollAlignAxisB=+Y  BaseAlignAxisB=+Z  RotationStandardAxis=+Z  RotationAngle=0  RotationAngleUnits=deg  RotationArbitraryAxis=[0 0 1]  RotationSequenceAxes=FollowerAxes  RotationSequence=XYX  RotationSequenceAngles=[0 0 0]  RotationSequenceAnglesUnits=deg  RotationMatrix=[1 0 0;0 1 0;0 0 1]  Quaternion=[1 0 0 0]  TranslationMethod=Cartesian  TranslationCartesianOffset=[0 0.254 0]  TranslationCartesianOffsetUnits=m  TranslationStandardAxis=+Z  TranslationStandardOffset=0  TranslationStandardOffsetUnits=m  TranslationROffset=0  TranslationROffsetUnits=m  TranslationThetaOffset=0  TranslationThetaOffsetUnits=deg  TranslationZOffset=0  TranslationZOffsetUnits=m
  Simulink-PS Converter : nesl_utility/Simulink-PS Converter  PhysicalDomain=network_engine_domain  SubClassName=ps_input  LeftPortType=input  RightPortType=output  PseudoPeriodic=off  Frequencies=[]  NoiseDistribution=none  NoiseParameters=[]  Unit=rad  AffineConversion=off  FilteringAndDerivatives=filter  SimscapeFilterOrder=2  InputFilterTimeConstant=0.001  UdotUserProvided=0
  Simulink-PS Converter1 : nesl_utility/Simulink-PS Converter  PhysicalDomain=network_engine_domain  SubClassName=ps_input  LeftPortType=input  RightPortType=output  PseudoPeriodic=off  Frequencies=[]  NoiseDistribution=none  NoiseParameters=[]  Unit=rad  AffineConversion=off  FilteringAndDerivatives=filter  SimscapeFilterOrder=2  InputFilterTimeConstant=0.001  UdotUserProvided=0
  Solver Configuration : nesl_utility/Solver Configuration  PhysicalDomain=network_engine_domain  SubClassName=solver  LeftPortType=input  RightPortType=generic  Tones=[]  Harmonics=[]  SimulateNoise=off  Profile=off  UseLocalSampling=off  EnableSwitchedLinearOptims=on  FrequencyDomain=off  UseCCode=off  RelTol=0.001  AbsTol=0.001  MinStep=1e-09  ToWorkspace=off  RevertToSquareIcSolve=off  NumHomotopyIterations=100  PhasorMode=off  PhasorModeNumHarmonics=1  ConsistencySolver=NEWTON_XTOL_AFTER_FTOL  IndexReductionMethod=DerivativeReplacement  DoDC=on  ResidualTolerance=1e-09  ConsistencyTolSource=GLOBAL  ConsistencyAbsTol=0.001  ConsistencyRelTol=0.001  ConsistencyTolFactor=0.001  UseLocalSolver=off  LocalSolverChoice=NE_BACKWARD_EULER_ADVANCER  ResolveIndetEquations=on  FunctionEvalNumThread=1  LocalSolverSampleTime=0.001  DoFixedCost=off  MaxNonlinIter=3  MaxModeIter=2  ComputeImpulses=off  ImpulseIterations=2  LinearAlgebra=auto  LinearAlgebraNumThread=0  EquationFormulation=NE_TIME_EF  DelaysMemoryBudget=1024  AutomaticFiltering=on  FilteringTimeConstant=0.001  PartitionStorageMethod=AS_NEEDED  PartitionMemoryBudget=1024  PartitionMethod=ROBUST  MultibodyUseLocalSolver=off  MultibodyLocalSolverChoice=ODE1  MultibodyLocalSolverSampleTime=0.001
  Transform Sensor : sm_lib/Frames and Transforms/Transform Sensor  MeasurementFrame=World  RotationSequence=XYX  SenseAngle=off  SenseAxis=off  SenseQ=off  SenseR=off  SenseRotationSequence=off  SenseOmegaX=off  SenseOmegaY=off  SenseOmegaZ=off  SenseOmega=off  SenseQDot=off  SenseRDot=off  SenseRotationSequenceDot=off  SenseAlphaX=off  SenseAlphaY=off  SenseAlphaZ=off  SenseAlpha=off  SenseQDDot=off  SenseRDDot=off  SenseX=on  SenseY=on  SenseZ=off  SenseXYZ=off  SenseRad=off  SenseAzim=off  SenseDist=off  SenseInc=off  SenseXDot=off  SenseYDot=off  SenseZDot=off  SenseXYZDot=off  SenseRadDot=off  SenseAzimDot=off  SenseDistDot=off  SenseIncDot=off  SenseXDDot=off  SenseYDDot=off  SenseZDDot=off  SenseXYZDDot=off  SenseRadDDot=off  SenseAzimDDot=off  SenseDistDDot=off  SenseIncDDot=off
  World Frame : sm_lib/Frames and Transforms/World Frame
  X : Outport
  Y : Outport  Port=2
  wires:
  theta/1 -> Simulink-PS Converter1/1
  phi/1 -> Simulink-PS Converter/1
  PS-Simulink Converter1/1 -> Y/1  "Y"
  PS-Simulink Converter/1 -> Gain1/1  "X"
  Gain1/1 -> X/1
  connections:
  World Frame/RConn1 -- Rigid Transform/LConn1 -- Transform Sensor/LConn1 -- Joint 1/LConn1 -- Solver Configuration/RConn1 -- Mechanism Configuration/RConn1
  Joint 3/LConn1 -- Link 2/RConn1
  Link 3/LConn1 -- Transform Sensor/RConn1 -- Joint 3/RConn1
  Simulink-PS Converter1/RConn1 -- Joint 5/LConn2
  Rigid Transform/RConn1 -- Joint 5/LConn1
  Link 3/RConn1 -- Joint 4/LConn1
  Link 1/RConn1 -- Joint 2/LConn1
  Link 4/LConn1 -- Joint 4/RConn1
  Link 4/RConn1 -- Joint 5/RConn1
  Link 2/LConn1 -- Joint 2/RConn1
  Link 1/LConn1 -- Joint 1/RConn1
  Simulink-PS Converter/RConn1 -- Joint 1/LConn2
  PS-Simulink Converter/LConn1 -- Transform Sensor/RConn2
  PS-Simulink Converter1/LConn1 -- Transform Sensor/RConn3

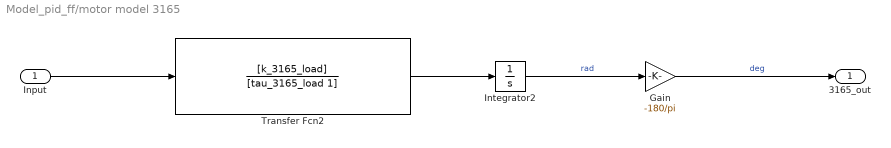
== system Model_pid_ff/motor model 3165 ==
  Input : Inport
  Gain : Gain  Gain=-180/pi
  Integrator2 : Integrator
  Transfer Fcn2 : TransferFcn  Numerator=[k_3165_load]  Denominator=[tau_3165_load 1]
  3165_out : Outport
  wires:
  Transfer Fcn2/1 -> Integrator2/1
  Input/1 -> Transfer Fcn2/1
  Integrator2/1 -> Gain/1  "rad"
  Gain/1 -> 3165_out/1  "deg"

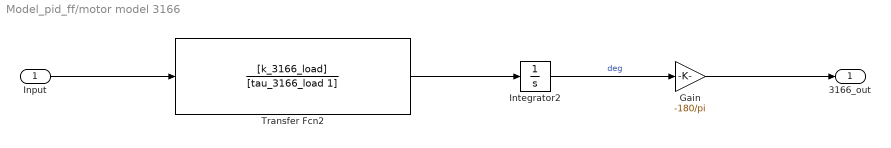
== system Model_pid_ff/motor model 3166 ==
  Input : Inport
  Gain : Gain  Gain=-180/pi
  Integrator2 : Integrator
  Transfer Fcn2 : TransferFcn  Numerator=[k_3166_load]  Denominator=[tau_3166_load 1]
  3166_out : Outport
  wires:
  Transfer Fcn2/1 -> Integrator2/1
  Input/1 -> Transfer Fcn2/1
  Integrator2/1 -> Gain/1  "deg"
  Gain/1 -> 3166_out/1

== matlab function Model_pid_ff/PID+FF 3166/MATLAB Function ==
  data: dtheta input; Vc_3166 parameter; w_eps parameter; y output
function y = friction_compensation(dtheta, Vc_3166, w_eps)
y = Vc_3166*tanh(dtheta/w_eps);

== matlab function Model_pid_ff/PID+FF 3165/MATLAB Function ==
  data: dphi input; Vc_3165 parameter; w_eps parameter; y output
function y = friction_compensation(dphi, Vc_3165, w_eps)
y = Vc_3165*tanh(dphi/w_eps);

== matlab function Model_pid_ff/direct kinematics ==
  data: phi input; xc output; theta input; yc output
function [xc, yc] = fcn(phi, theta)
l = 0.127;
a = 2 - sin(theta) - cos(phi);
b = cos(theta) - sin(phi);
s = sqrt(a^2 + b^2);
h = l*sqrt(1 - s^2/4);

% Nonlinear forward kinematics of point C
xc = l/2*(2 - sin(theta) + cos(phi)) - h*b/s;
yc = l/2*(cos(theta) + sin(phi))     + h*a/s;

== matlab function Model_pid_ff/square trajectory ==
  data: x output; t input; y output; vx output; vy output; ax output; ay output
% function [x, y, vx, vy, ax, ay] = square_gen_smooth(t)
% c  = [0.127; 0.127];
% s  = 0.09;
% T  = 4;
% Ts = T/4;
% P = [c(1)-s/2, c(1)+s/2, c(1)+s/2, c(1)-s/2, c(1)-s/2;
%      c(2)-s/2, c(2)-s/2, c(2)+s/2, c(2)+s/2, c(2)-s/2];
% 
% tau = mod(t, T) / Ts;
% k   = min(floor(tau), 3);
% f   = tau - k;
% 
% % quintic time scaling and its derivatives w.r.t. real time
% sig   = 10*f^3 - 15*f^4 + 6*f^5;
% dsig  = (30*f^2 - 60*f^3 + 30*f^4) / Ts;
% ddsig = (60*f - 180*f^2 + 120*f^3) / Ts^2;
% 
% dx = P(1,k+2) - P(1,k+1);
% dy = P(2,k+2) - P(2,k+1);
% 
% x  = P(1,k+1) + sig*dx;     y  = P(2,k+1) + sig*dy;
% vx = dsig*dx;               vy = dsig*dy;
% ax = ddsig*dx;              ay = ddsig*dy;
% end

function [x, y, vx, vy, ax, ay] = square_gen_smooth(t)
% SQUARE_GEN_SMOOTH  Square path for the tip C (counter-clockwise), with a step at the start.
%   t <  t_hold : hold the start point Q (zero speed and acceleration -> zero feedforward).
%                 The robot starts at home = centre c, so this is a STEP for the loop.
%   t >= t_hold : laps Q -> 4 corners -> Q, each segment with a quintic time scaling
%                 (zero speed and acceleration at both ends).
% Q is the midpoint of one side (the closest points of the square to home, s/2 away).
% Joint move of the step:  East/West -> mostly motor 3166,  North/South -> mostly motor 3165.

%% Settings
c      = [0.127; 0.127];   % [m] centre of the square = home position of the tip
s      = 0.09;             % [m] side
T      = 4;                % [s] time of one lap
t_hold = 1.5;              % [s] time spent at Q before the laps
start  = 1;                % start side: 1 = East, 2 = North, 3 = West, 4 = South

%% Waypoints of one lap
h = s/2;
corners = c + [-h,  h,  h, -h;            % SW, SE, NE, NW  (counter-clockwise)
               -h, -h,  h,  h];
first   = [3, 4, 1, 2];                   % first corner reached from each side: E->NE, N->NW, W->SW, S->SE
order   = circshift(corners, -(first(start) - 1), 2);   % the 4 corners, starting from that one
Q       = (order(:, 4) + order(:, 1))/2;  % midpoint of the start side (between last and first corner)
W       = [Q, order, Q];                  % 6 waypoints -> 5 segments

dur = T/4*[0.5, 1, 1, 1, 0.5];            % [s] segment durations (half sides at both ends)
t0  = [0, cumsum(dur)];                   % [s] start time of each segment inside a lap

%% Phase 1: step to Q and hold
if t < t_hold
    x = Q(1);  y = Q(2);  vx = 0;  vy = 0;  ax = 0;  ay = 0;
    return
end

%% Phase 2: laps
tl = mod(t - t_hold, T);                  % time inside the lap
k  = 1 + sum(tl >= t0(2:5));              % current segment (1..5)
Tk = dur(k);
f  = (tl - t0(k))/Tk;                     % 0 -> 1 along the segment

sig   = 10*f^3 - 15*f^4 + 6*f^5;                % quintic: position fraction
dsig  = (30*f^2 - 60*f^3 + 30*f^4)/Tk;          % its time derivative
ddsig = (60*f - 180*f^2 + 120*f^3)/Tk^2;        % its second time derivative

d  = W(:, k+1) - W(:, k);                 % segment vector
x  = W(1, k) + sig*d(1);    y  = W(2, k) + sig*d(2);
vx = dsig*d(1);             vy = dsig*d(2);
ax = ddsig*d(1);            ay = ddsig*d(2);
end

== matlab function Model_pid_ff/circle trajectory ==
  data: x output; t input; y output; vx output; vy output; ax output; ay output
function [x, y, vx, vy, ax, ay] = circle_gen_smooth(t)
% The circle is inscribed in the square (same center, diameter = side).
c   = [0.127; 0.127];   % center [m]
s   = 0.09;             % side of the square [m]
r   = s/2;              % radius [m]
T   = 4;                % duration of one lap [s]
th0 = 5*pi/4;           % starting angle: bottom-left, like the square

% quintic time scaling on the angle: one full lap in T seconds,
% with zero velocity and acceleration at the start and end of each lap
f     = mod(t, T) / T;                              % normalized time 0..1
sig   = 10*f^3 - 15*f^4 + 6*f^5;
dsig  = (30*f^2 - 60*f^3 + 30*f^4) / T;
ddsig = (60*f - 180*f^2 + 120*f^3) / T^2;

th   = th0 + 2*pi*sig;      % angle on the circle [rad]
dth  = 2*pi*dsig;           % angular velocity [rad/s]
ddth = 2*pi*ddsig;          % angular acceleration [rad/s^2]

% position, velocity and acceleration (chain rule)
x  = c(1) + r*cos(th);
y  = c(2) + r*sin(th);
vx = -r*sin(th)*dth;
vy =  r*cos(th)*dth;
ax = -r*cos(th)*dth^2 - r*sin(th)*ddth;   % centripetal + tangential
ay = -r*sin(th)*dth^2 + r*cos(th)*ddth;
end

== matlab function Model_pid_ff/inverse kinematics ==
  data: x input; phi output; y input; theta output; vx input; vy input; ax input; ay input; dphi output; dtheta output; ddphi output; ddtheta output
function [phi, theta, dphi, dtheta, ddphi, ddtheta] = fcn(x, y, vx, vy, ax, ay)
% Inverse kinematics + joint velocity/acceleration, self-contained.
l = 0.127;

persistent q0
if isempty(q0)
    q0 = [0; 0];                 % home configuration
end

% ---- position IK (damped Newton, warm-started from previous step) ----
q = q0;
p_des   = [x; y];
maxIter = 50;
tol     = 1e-9;
lambda  = 1e-10;
for k = 1:maxIter
    p   = FK(q(1), q(2), l);
    err = p - p_des;
    if norm(err) < tol
        break
    end
    J  = jac(q, l);
    dq = -(J.'*J + lambda*eye(2)) \ (J.'*err);
    st = 1;
    for m = 1:10
        qn = q + st*dq;
        if norm(FK(qn(1), qn(2), l) - p_des) < norm(err)
            break
        end
        st = st/2;
    end
    q = q + st*dq;
end
q0 = q;                          % warm start for next call
phi   = q(1);
theta = q(2);

% ---- velocity and acceleration ----
J  = jac(q, l);
qd = J \ [vx; vy];

e    = 1e-4;
Jdot = (jac(q + e*qd, l) - jac(q - e*qd, l)) / (2*e);
qdd  = J \ ([ax; ay] - Jdot*qd);

dphi   = qd(1);   dtheta  = qd(2);
ddphi  = qdd(1);  ddtheta = qdd(2);
end

function J = jac(q, l)
h = 1e-6;
J = zeros(2,2);
for j = 1:2
    d = zeros(2,1);
    d(j) = h;
    J(:,j) = (FK(q(1)+d(1), q(2)+d(2), l) - FK(q(1)-d(1), q(2)-d(2), l)) / (2*h);
end
end

function p = FK(phi, theta, l)
a = 2 - sin(theta) - cos(phi);
b = cos(theta) - sin(phi);
s = sqrt(a^2 + b^2);
s = max(s, 1e-9);
h = l * sqrt(max(1 - s^2/4, 0));
xc = l/2*(2 - sin(theta) + cos(phi)) - h*b/s;
yc = l/2*(cos(theta) + sin(phi))     + h*a/s;
p  = [xc; yc];
end
